simulink model "E8_SimulinkMIMOSys"  (R2024a)
settings: Solver=VariableStepAuto  StartTime=0.0  StopTime=10.0  RelTol=1e-3
settings Model: Creator=Sanagostar  LastModifiedBy=Sanagostar

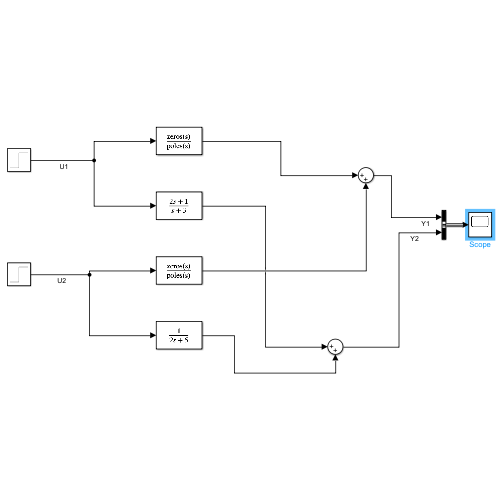
[thumbnail: Simulink's stored preview of the top-level diagram]
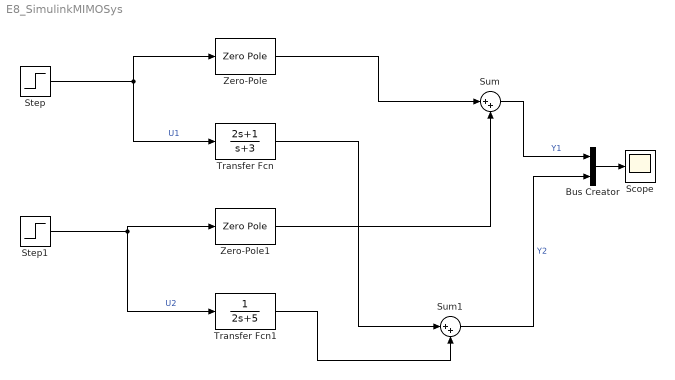
== system E8_SimulinkMIMOSys ==
  Bus Creator : BusCreator  Inputs=2
  Scope : Scope
  Step : Step  SampleTime=0
  Step1 : Step  Time=5  SampleTime=0
  Sum : Sum  Inputs=|++
  Sum1 : Sum  Inputs=|++
  Transfer Fcn : TransferFcn  Numerator=[2 1]  Denominator=[1 3]
  Transfer Fcn1 : TransferFcn  Denominator=[2 5]
  Zero-Pole : ZeroPole  Zeros=[]  Poles=[-1]
  Zero-Pole1 : ZeroPole  Poles=[-2]
  wires:
  Step/1 -> Transfer Fcn/1, Zero-Pole/1  "U1"
  Step1/1 -> Transfer Fcn1/1, Zero-Pole1/1  "U2"
  Zero-Pole/1 -> Sum/1
  Zero-Pole1/1 -> Sum/2
  Transfer Fcn/1 -> Sum1/1
  Transfer Fcn1/1 -> Sum1/2
  Sum1/1 -> Bus Creator/2  "Y2"
  Sum/1 -> Bus Creator/1  "Y1"
  Bus Creator/1 -> Scope/1
